simulink model "ex_03_sim"  (R2024b)
settings: Solver=VariableStepAuto  StartTime=0.0  StopTime=10.0  RelTol=1e-3
values from neighbouring files (symbols this model uses):
  A = d.A    [ex_03_main.m]
  A_v = d.A_v    [ex_03_main.m]
  B = d.B    [ex_03_main.m]
  c = d.c(:).'    [ex_03_main.m]
  C = d.C    [ex_03_main.m]
  D = d.D    [ex_03_main.m]
  Initial_v = d.Initial_v(:)    [ex_03_main.m]
undefined symbols (not defined in the file or in its folder): B_v, C_v, D_v, k_v, k_x, r
settings Model: Creator=54238  LastModifiedBy=54238

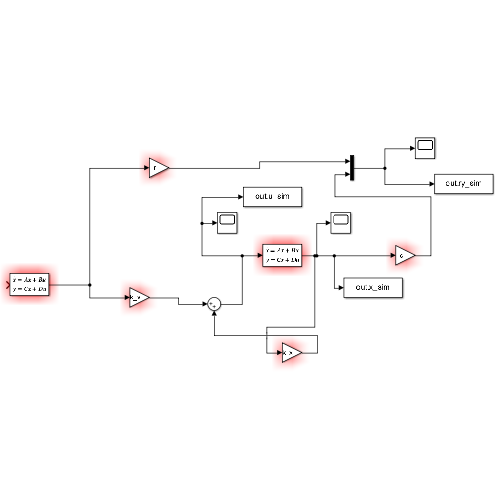
[thumbnail: Simulink's stored preview of the top-level diagram]
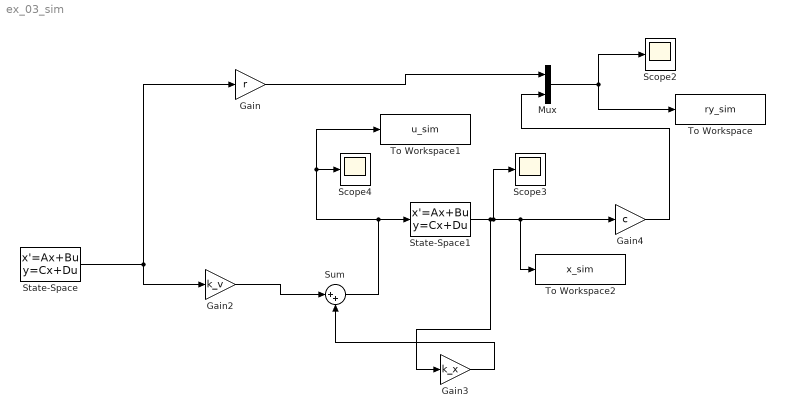
== system ex_03_sim ==
  Gain : Gain  Gain=r
  Gain2 : Gain  Gain=k_v
  Gain3 : Gain  Gain=k_x
  Gain4 : Gain  Gain=c
  Mux : Mux  Inputs=2
  Scope2 : Scope
  Scope3 : Scope
  Scope4 : Scope
  State-Space : StateSpace  A=A_v  B=B_v  C=C_v  D=D_v  InitialCondition=Initial_v
  State-Space1 : StateSpace  A=A  B=B  C=C  D=D  InitialCondition=0
  Sum : Sum  Inputs=|++
  To Workspace : ToWorkspace  VariableName=ry_sim  SaveFormat=Timeseries  SampleTime=-1
  To Workspace1 : ToWorkspace  VariableName=u_sim  SaveFormat=Timeseries  SampleTime=-1
  To Workspace2 : ToWorkspace  VariableName=x_sim  SaveFormat=Timeseries  SampleTime=-1
  wires:
  State-Space/1 -> Gain/1, Gain2/1
  Gain/1 -> Mux/1
  State-Space1/1 -> Gain3/1, To Workspace2/1, Gain4/1, Scope3/1
  Gain2/1 -> Sum/1
  Sum/1 -> To Workspace1/1, Scope4/1, State-Space1/1
  Gain4/1 -> Mux/2
  Mux/1 -> To Workspace/1, Scope2/1
  Gain3/1 -> Sum/2
